simulink model "HybridShip_ModelE_PlantStepE_Stream"  (R2026a)
settings: Solver=ode3  StopTime=7200  FixedStep=0.01
undefined symbols (not defined in the file): ADAPTER_FORCE_MODE, ADAPTER_FORCE_P1_KW, ADAPTER_FORCE_P2_KW, ASSUMED_C_bus, ASSUMED_Drive_TimeConstant, ASSUMED_eta_dcdc, ASSUMED_eta_rect, ASSUMED_K_droop, ASSUMED_SOC_ChgDerate_Start, ASSUMED_SOC_DisDerate_Start, ASSUMED_SOC_max, ASSUMED_SOC_min, ASSUMED_SpeedPI_Ki, ASSUMED_SpeedPI_Kp, ASSUMED_V_floor, Bat_C1_LUT_F, Bat_eta_coul, Bat_I_limit_surrogate_A, Bat_OCV_LUT_V, Bat_P_conv_bus_max_kW, Bat_Q_nom_Ah, Bat_R0_chg_mult, Bat_R0_LUT_ohm, Bat_R1_LUT_ohm, Bat_SOC_init, Bat_SOC_LUT_nodes, Bat_V_max_V, Bat_V_min_V, CCS_Vdc_Steady_Band, CCS_Vdc_Transient_Band, DG_BSFC_gkWh, DG_BSFC_P_kW, DG_C_start_kg, DG_P_min_kW, DG_P_rated_kW, DG_ramp_kW_per_s, DG_t_starting_s, DG_t_sync_s, DG_tau_s, DiscIntNeverNeededParam, Elec_Eff, F_env_const, Gear_Eff, Gear_Ratio, Hull_k_form, Hull_K_R, Hull_Lpp_m, Hull_T_m, K_Fv, K_Fw, K_Qv, K_Qw, Manual_Cmd_RateLimit_kW_per_s, Mot_P_nom, Mot_T_max, N_ticks_cooldown, N_ticks_starting, N_ticks_sync, nu_water, omega_min_radps ... (+40)
libraries: simulink x6
(part 2 of 2)

== matlab function HybridShip_ModelE_PlantStepE_Stream/06_Genset_System/GensetUnitE_DG1 ==
  settings: updateMethod=DISCRETE  sampleTime=0.01
  data: cmd_start input; P_actual_kW output; cmd_stop input; P_ref_kW input; state output; below_min_flag output; start_count output; DG_P_rated_kW parameter; DG_P_min_kW parameter; DG_ramp_kW_per_s parameter; DG_tau_s parameter; N_ticks_starting parameter; N_ticks_sync parameter; N_ticks_cooldown parameter; Pgen_init parameter
function [P_actual_kW, state, below_min_flag, start_count] = GensetUnitE(...
    cmd_start, cmd_stop, P_ref_kW, ...
    DG_P_rated_kW, DG_P_min_kW, DG_ramp_kW_per_s, DG_tau_s, ...
N_ticks_starting, N_ticks_sync, N_ticks_cooldown, Pgen_init)
%#codegen
% GensetUnitE：单发电机组启停状态机 + 功率链（Model E, FR-418/419, OQ-6 定稿）
%   DG1/DG2 各用一个块实例（同一代码）；固定步 0.01 s，每步调用一次 = 1 tick；
%   状态驻留用整数 tick 计数做转移判据（OQ-6，禁止浮点时间比较）。
%   state: 0=OFF 1=STARTING 2=SYNCHRONIZING 3=ON 4=COOLDOWN（数值状态，供 fuel/log 用）
%   D-4：min up/min down time 不在本 Plant 内（unit commitment 属 B 包 PMS v2）；
%        COOLDOWN 物理驻留 N_ticks_cooldown 表达停机间隔，期间 cmd_start 忽略。
%   aborted-start：STARTING/SYNC 不可中断；cmd_stop 只置 pending_stop，进入 ON 后一拍内执行停机。
%   OFF 态 stop 优先（2026-09-04 主 Agent 裁决）：cmd_start=1 且 cmd_stop=1 时保持 OFF，防停机后无限再启动。
persistent st n_tick pending_stop n_starts P_ramp P_lag
if isempty(st)
    st = 0;                 % 初始 OFF（新状态机初始 OFF；Pgen_init 仅作 P_lag legacy 初值）
    n_tick = 0;             % 当前状态驻留 tick 计数
    pending_stop = false;   % STARTING/SYNC 期间登记的停机请求
    n_starts = 0;           % 完成启动次数（SYNC 完成时 +1，含 aborted-start）
    P_ramp = 0;             % 爬坡状态 [kW]
    P_lag = Pgen_init;      % 一阶惯性状态 [kW]（legacy 常开模型初值兼容语义）
end

P_actual_kW = 0;            % 非 ON 态恒 0；ON 态由功率链覆写
below_min_flag = 0;         % 仅 ON 态置位（ref < P_min；switch 后按最终状态统一判定）

switch st
    case 0 % OFF：cmd_start 触发启动（cmd_stop 有效时 stop 优先，防停机后无限再启动）
        if cmd_start > 0.5 && cmd_stop < 0.5
            st = 1;                  % OFF -> STARTING
            n_tick = 0;
            pending_stop = false;    % n_starts 不在此刻加（SYNC 完成时才计）
            P_ramp = 0;              % 启动从零爬坡
            P_lag = 0;
        end

    case 1 % STARTING：不可中断（aborted-start 只登记）
        n_tick = n_tick + 1;
        if cmd_stop > 0.5
            pending_stop = true;
        end
        if n_tick >= N_ticks_starting
            st = 2;                  % STARTING -> SYNCHRONIZING
            n_tick = 0;
        end

    case 2 % SYNCHRONIZING：不可中断
        n_tick = n_tick + 1;
        if cmd_stop > 0.5
            pending_stop = true;
        end
        if n_tick >= N_ticks_sync
            n_starts = n_starts + 1; % 启动完成（启动燃油由此计量一次）
            st = 3;                  % SYNCHRONIZING -> ON
            n_tick = 0;
        end

    case 3 % ON：功率链 + 停机命令（pending_stop 在此执行）
        if cmd_stop > 0.5 || pending_stop
            pending_stop = false;
            st = 4;                  % ON -> COOLDOWN（断路器分闸，本拍 P=0）
            n_tick = 0;
        else
            % ref clamp [P_min, rated]（below_min_flag 在 switch 后按最终状态统一置位）
            P_ref_c = min(max(P_ref_kW, DG_P_min_kW), DG_P_rated_kW);
            if P_ramp < P_ref_c
                P_ramp = min(P_ramp + DG_ramp_kW_per_s*0.01, P_ref_c);  % 爬坡限幅（0.01 s 步）
            elseif P_ramp > P_ref_c
                P_ramp = max(P_ramp - DG_ramp_kW_per_s*0.01, P_ref_c);
            end
            P_lag = P_lag + (P_ramp - P_lag)*0.01/DG_tau_s;             % 一阶惯性 tau
            P_actual_kW = min(max(P_lag, 0), DG_P_rated_kW);
            % 注：爬坡过渡期 P<P_min 为 registered 过渡（below_min_flag 登记；
            % 燃油侧按 clamp 到 BSFC 下节点(125)查表，见 FuelModelE）
        end

    case 4 % COOLDOWN：P=0；cmd_start 忽略（D-4：物理驻留表达最小停机间隔）
        n_tick = n_tick + 1;
        if n_tick >= N_ticks_cooldown
            st = 0;                  % COOLDOWN -> OFF
            n_tick = 0;
        end

    otherwise % 防御：非法状态归 OFF（无 NaN 路径）
        st = 0;
        n_tick = 0;
end

state = st;                  % 输出为本拍转移后的状态
if st == 3 && P_ref_kW < DG_P_min_kW
    below_min_flag = 1;      % 输出约定：flag=1 当且仅当 state==3 且 ref<P_min（含 ON 入口拍）
end
start_count = n_starts;
end

== matlab function HybridShip_ModelE_PlantStepE_Stream/06_Genset_System/GensetUnitE_DG2 ==
  settings: updateMethod=DISCRETE  sampleTime=0.01
  data: cmd_start input; P_actual_kW output; cmd_stop input; P_ref_kW input; state output; below_min_flag output; start_count output; DG_P_rated_kW parameter; DG_P_min_kW parameter; DG_ramp_kW_per_s parameter; DG_tau_s parameter; N_ticks_starting parameter; N_ticks_sync parameter; N_ticks_cooldown parameter; Pgen_init parameter
function [P_actual_kW, state, below_min_flag, start_count] = GensetUnitE(...
    cmd_start, cmd_stop, P_ref_kW, ...
    DG_P_rated_kW, DG_P_min_kW, DG_ramp_kW_per_s, DG_tau_s, ...
N_ticks_starting, N_ticks_sync, N_ticks_cooldown, Pgen_init)
%#codegen
% GensetUnitE：单发电机组启停状态机 + 功率链（Model E, FR-418/419, OQ-6 定稿）
%   DG1/DG2 各用一个块实例（同一代码）；固定步 0.01 s，每步调用一次 = 1 tick；
%   状态驻留用整数 tick 计数做转移判据（OQ-6，禁止浮点时间比较）。
%   state: 0=OFF 1=STARTING 2=SYNCHRONIZING 3=ON 4=COOLDOWN（数值状态，供 fuel/log 用）
%   D-4：min up/min down time 不在本 Plant 内（unit commitment 属 B 包 PMS v2）；
%        COOLDOWN 物理驻留 N_ticks_cooldown 表达停机间隔，期间 cmd_start 忽略。
%   aborted-start：STARTING/SYNC 不可中断；cmd_stop 只置 pending_stop，进入 ON 后一拍内执行停机。
%   OFF 态 stop 优先（2026-09-04 主 Agent 裁决）：cmd_start=1 且 cmd_stop=1 时保持 OFF，防停机后无限再启动。
persistent st n_tick pending_stop n_starts P_ramp P_lag
if isempty(st)
    st = 0;                 % 初始 OFF（新状态机初始 OFF；Pgen_init 仅作 P_lag legacy 初值）
    n_tick = 0;             % 当前状态驻留 tick 计数
    pending_stop = false;   % STARTING/SYNC 期间登记的停机请求
    n_starts = 0;           % 完成启动次数（SYNC 完成时 +1，含 aborted-start）
    P_ramp = 0;             % 爬坡状态 [kW]
    P_lag = Pgen_init;      % 一阶惯性状态 [kW]（legacy 常开模型初值兼容语义）
end

P_actual_kW = 0;            % 非 ON 态恒 0；ON 态由功率链覆写
below_min_flag = 0;         % 仅 ON 态置位（ref < P_min；switch 后按最终状态统一判定）

switch st
    case 0 % OFF：cmd_start 触发启动（cmd_stop 有效时 stop 优先，防停机后无限再启动）
        if cmd_start > 0.5 && cmd_stop < 0.5
            st = 1;                  % OFF -> STARTING
            n_tick = 0;
            pending_stop = false;    % n_starts 不在此刻加（SYNC 完成时才计）
            P_ramp = 0;              % 启动从零爬坡
            P_lag = 0;
        end

    case 1 % STARTING：不可中断（aborted-start 只登记）
        n_tick = n_tick + 1;
        if cmd_stop > 0.5
            pending_stop = true;
        end
        if n_tick >= N_ticks_starting
            st = 2;                  % STARTING -> SYNCHRONIZING
            n_tick = 0;
        end

    case 2 % SYNCHRONIZING：不可中断
        n_tick = n_tick + 1;
        if cmd_stop > 0.5
            pending_stop = true;
        end
        if n_tick >= N_ticks_sync
            n_starts = n_starts + 1; % 启动完成（启动燃油由此计量一次）
            st = 3;                  % SYNCHRONIZING -> ON
            n_tick = 0;
        end

    case 3 % ON：功率链 + 停机命令（pending_stop 在此执行）
        if cmd_stop > 0.5 || pending_stop
            pending_stop = false;
            st = 4;                  % ON -> COOLDOWN（断路器分闸，本拍 P=0）
            n_tick = 0;
        else
            % ref clamp [P_min, rated]（below_min_flag 在 switch 后按最终状态统一置位）
            P_ref_c = min(max(P_ref_kW, DG_P_min_kW), DG_P_rated_kW);
            if P_ramp < P_ref_c
                P_ramp = min(P_ramp + DG_ramp_kW_per_s*0.01, P_ref_c);  % 爬坡限幅（0.01 s 步）
            elseif P_ramp > P_ref_c
                P_ramp = max(P_ramp - DG_ramp_kW_per_s*0.01, P_ref_c);
            end
            P_lag = P_lag + (P_ramp - P_lag)*0.01/DG_tau_s;             % 一阶惯性 tau
            P_actual_kW = min(max(P_lag, 0), DG_P_rated_kW);
            % 注：爬坡过渡期 P<P_min 为 registered 过渡（below_min_flag 登记；
            % 燃油侧按 clamp 到 BSFC 下节点(125)查表，见 FuelModelE）
        end

    case 4 % COOLDOWN：P=0；cmd_start 忽略（D-4：物理驻留表达最小停机间隔）
        n_tick = n_tick + 1;
        if n_tick >= N_ticks_cooldown
            st = 0;                  % COOLDOWN -> OFF
            n_tick = 0;
        end

    otherwise % 防御：非法状态归 OFF（无 NaN 路径）
        st = 0;
        n_tick = 0;
end

state = st;                  % 输出为本拍转移后的状态
if st == 3 && P_ref_kW < DG_P_min_kW
    below_min_flag = 1;      % 输出约定：flag=1 当且仅当 state==3 且 ref<P_min（含 ON 入口拍）
end
start_count = n_starts;
end

== matlab function HybridShip_ModelE_PlantStepE_Stream/07_PMS_v2/PMS_Demand_Policy ==
  settings: updateMethod=DISCRETE  sampleTime=0.01
  data: P_load_gen_kW input; P_gen_req_baseline_kW output; SOC input; N_dispatch_fb input; P_commit_kW output; u_recovery output; P_recovery_actual_kW output; PMS_LoadLPF_tau_s parameter double size=1; PMS_SOC_lo parameter double size=1; PMS_SOC_recovered parameter double size=1; PMS_P_chg_recovery_kW parameter double size=1; DG_P_rated_kW parameter double size=1
function [P_gen_req_baseline_kW, P_commit_kW, u_recovery, P_recovery_actual_kW] = PMSDemandPolicyE(P_load_gen_kW, SOC, N_dispatch_fb, PMS_LoadLPF_tau_s, PMS_SOC_lo, PMS_SOC_recovered, PMS_P_chg_recovery_kW, DG_P_rated_kW)
%#codegen
% PMSDemandPolicyE：Baseline_Demand_Policy 发电需求律（Model E Phase 4-B, FR-432~435, T-002 链 A）
%   依据：.specs/phase4-b-pms-safety/design.md §5.3 + requirements FR-432/433/434/435（AC-417）；
%   brainstorm D-B3（Demand Policy 四数冻结）/ D-B4（P_commit 信号语义方案 b）/ D-B6 / D-B14。
%   角色：07_PMS_v2 内 Baseline source（ems_health_ok=0 时的确定性热备份，D-B7 ③）；
%   advanced EMS source 的 P_gen_req=P_EMS 直送不削减（FR-434），削减只发生在本 Baseline source 内部。
%
%   canonical 功率域（DD-1，genset-side generator-equivalent）：
%     - 全部输入/输出量均为 genset-side generator-equivalent；P_load_gen_kW 已在 07_PMS_v2
%       输入边界经 X_b2g_* 由 bus 侧 ÷ASSUMED_eta_rect 换算入域，本块零换算直用；
%     - PMS_P_chg_recovery_kW=100 kW 为 generator-equivalent recovery bias（≈bus 侧新增发电
%       约 97 kW），禁止表述为"电池 100 kW 实际充电"（DD-1 措辞纪律）。
%
%   输入：P_load_gen_kW 负荷（generator-equivalent）；SOC [-]；N_dispatch_fb dispatch 反馈
%     （在线机组数，**上一拍语义由调用方 UnitDelay 保证**——本函数直接消费当拍入参，
%     内部不再延迟，design §5.3）；PMS_LoadLPF_tau_s / PMS_SOC_lo / PMS_SOC_recovered /
%     PMS_P_chg_recovery_kW 为 FR-435 四参数（全 ENGINEERING_SURROGATE，数值事实源
%     config/ModelE_Control_Parameters.m，敏感性 τ∈{30,120} 冻结登记不扫）；DG_P_rated_kW
%     单机额定（genset 域字面，DD-1）。
%   输出：P_gen_req_baseline_kW = LPF(P_load) + P_recovery_actual（FR-432）；
%     P_commit_kW = LPF(P_load)（commitment 判据信号，不含 recovery 偏置，D-B4 方案 b）；
%     u_recovery SOC 滞回状态（供 logging，design §5.3）；P_recovery_actual_kW 实际恢复偏置。
%
%   离散约定：固定步 0.01 s，每调用一次 = 1 tick；dt=0.01 硬编码于 LPF 更新，
%   若模型固定步长变更须一并重推（同 GensetUnitE OQ-6 口径）。
%   纯 MATLAB：persistent 为唯一状态载体；无 toolbox 依赖；无 evalin/assignin/全局变量。

persistent P_load_filt u_rec
% 注：R2026a MATLAB Function 块解析纪律——persistent 变量不得直接作为输出参量，
% 故滞回状态本体为 u_rec，输出名 u_recovery 在每拍末拷贝输出（语义不变）。
if isempty(P_load_filt)
    P_load_filt = P_load_gen_kW;    % y[0]=x[0]（design §5.3；首拍 LPF 更新数值恒等）
    u_rec = false;                  % FR-433 初值 false
end

% (1) 一阶 LPF 前向欧拉（FR-432）：y[k]=y[k-1]+(Ts/τ)(x[k]-y[k-1])，τ=PMS_LoadLPF_tau_s
%     前向欧拉**非双线性**；标称 τ=60 s 时 Ts/τ≈1.67e-4，远在 0<Ts/τ<2 稳定界内、稳定裕量大
%     （禁称"无条件稳定"，design §5.3 措辞纪律）。
P_load_filt = P_load_filt + (0.01/PMS_LoadLPF_tau_s)*(P_load_gen_kW - P_load_filt);

% (2) SOC 滞回（FR-433，比较符号冻结；D-B3）：<=PMS_SOC_lo 进 / >=PMS_SOC_recovered 出 / 其间保持
if SOC <= PMS_SOC_lo
    u_rec = true;
elseif SOC >= PMS_SOC_recovered
    u_rec = false;
end
u_recovery = u_rec;                 % 输出本拍评估后的滞回状态（供 logging，design §5.3）

% (3) 恢复偏置（FR-434 non-firm/opportunistic）：负荷服务优先，削减只在 Baseline source 内部
%     （recovery 不得单独触发 DG2 启动——commitment 判据用 P_commit_kW，D-B4 结构性规则；
%       EMS 直送不削减，指令/功率 mismatch 经 dispatch 诊断量暴露，D-B6/D-B14）
P_recovery_actual_kW = double(u_rec) * max(0, min(PMS_P_chg_recovery_kW, ...
    DG_P_rated_kW*N_dispatch_fb - P_load_filt));

% (4) 基线发电需求 = LPF(P_load) + 实际恢复偏置（FR-432 / design §5.3）
P_gen_req_baseline_kW = P_load_filt + P_recovery_actual_kW;

% (5) commitment 判据信号 = LPF(P_load)，不含 recovery 偏置（D-B4 方案 b：
%     恢复充电为 opportunistic/non-firm 需求，不得影响启停门槛判定）
P_commit_kW = P_load_filt;
end

== stateflow chart HybridShip_ModelE_PlantStepE_Stream/07_PMS_v2/PMS_Commitment_Supervisor ==
  settings: updateMethod=DISCRETE  sampleTime=0.01
  state ONE_DG_NORMAL
    entry: if (commitment_state == 0)
    commitment_state = 1;
    reason_code = 0;
    audit_valid = 0;
    start_hold_timer = 0; stop_hold_timer = 0; online_timer = 0;
    cmd_onoff_DG1 = double(fault_latch_DG1 < 0.5);
    cmd_onoff_DG2 = 0;
    else
    audit_old_state = commitment_state; audit_new_state = 1;
    audit_P_commit_kW = P_commit_kW;
    audit_t_start_hold = start_hold_timer; audit_t_stop_hold = stop_hold_timer;
    audit_t_online = online_timer;
    audit_safety_override = double(tr_reason >= 3);
    audit_valid = 1;
    reason_code = tr_reason;
    commitment_state = 1;
    start_hold_timer = 0; stop_hold_timer = 0; online_timer = 0;
    cmd_onoff_DG1 = double(fault_latch_DG1 < 0.5);
    cmd_onoff_DG2 = 0;
    end
    during: cmd_onoff_DG1 = double(fault_latch_DG1 < 0.5);
    cmd_onoff_DG2 = 0;
    stop_hold_timer = 0; online_timer = 0;
    if (P_commit_kW > PMS_start_threshold_kW)
    start_hold_timer = min(start_hold_timer + 1, T_start_hold_ticks);
    else
    start_hold_timer = 0;
    end
  state DG2_START_PENDING
    entry: audit_old_state = commitment_state; audit_new_state = 2;
    audit_P_commit_kW = P_commit_kW;
    audit_t_start_hold = start_hold_timer; audit_t_stop_hold = stop_hold_timer;
    audit_t_online = online_timer;
    audit_safety_override = double(tr_reason >= 3);
    audit_valid = 1;
    reason_code = tr_reason; pending_reason = tr_reason;
    commitment_state = 2;
    start_hold_timer = 0; stop_hold_timer = 0; online_timer = 0;
    cmd_onoff_DG1 = double(fault_latch_DG1 < 0.5);
    cmd_onoff_DG2 = double(fault_latch_DG2 < 0.5);
    during: cmd_onoff_DG1 = double(fault_latch_DG1 < 0.5);
    cmd_onoff_DG2 = double(fault_latch_DG2 < 0.5);
    start_hold_timer = 0; stop_hold_timer = 0; online_timer = 0;
  state TWO_DG_NORMAL
    entry: audit_old_state = commitment_state; audit_new_state = 3;
    audit_P_commit_kW = P_commit_kW;
    audit_t_start_hold = start_hold_timer; audit_t_stop_hold = stop_hold_timer;
    audit_t_online = online_timer;
    audit_safety_override = double(tr_reason >= 3);
    audit_valid = 1;
    reason_code = tr_reason;
    commitment_state = 3;
    start_hold_timer = 0; stop_hold_timer = 0; online_timer = 0;
    cmd_onoff_DG1 = double(fault_latch_DG1 < 0.5);
    cmd_onoff_DG2 = double(fault_latch_DG2 < 0.5);
    during: cmd_onoff_DG1 = double(fault_latch_DG1 < 0.5);
    cmd_onoff_DG2 = double(fault_latch_DG2 < 0.5);
    start_hold_timer = 0;
    if (P_commit_kW < PMS_stop_threshold_kW)
    stop_hold_timer = min(stop_hold_timer + 1, T_stop_hold_ticks);
    else
    stop_hold_timer = 0;
    end
    if (state_DG2 == 3)
    online_timer = min(online_timer + 1, PMS_min_up_ticks);
    else
    online_timer = 0;
    end
  DG2_START_PENDING -> ONE_DG_NORMAL [order 1] : [fault_latch_DG2 > 0.5]{tr_reason = 3;}
  TWO_DG_NORMAL -> ONE_DG_NORMAL [order 1] : [fault_latch_DG2 > 0.5]{tr_reason = 3;}
  TWO_DG_NORMAL -> ONE_DG_NORMAL [order 2] : [force_stop_dg2_req > 0.5]{tr_reason = force_stop_reason;}
  TWO_DG_NORMAL -> ONE_DG_NORMAL [order 3] : [P_commit_kW < PMS_stop_threshold_kW && stop_hold_timer >= T_stop_hold_ticks && online_timer >= PMS_min_up_ticks]{tr_reason = 2;}
  (default) -> ONE_DG_NORMAL : {tr_reason = 0;}
  ONE_DG_NORMAL -> DG2_START_PENDING [order 1] : [force_start_dg2_req > 0.5 && fault_latch_DG2 < 0.5]{tr_reason = force_start_reason;}
  ONE_DG_NORMAL -> DG2_START_PENDING [order 2] : [start_hold_timer >= T_start_hold_ticks && fault_latch_DG2 < 0.5]{tr_reason = 1;}
  DG2_START_PENDING -> TWO_DG_NORMAL [order 2] : [state_DG2 == 3]{tr_reason = pending_reason;}
  data: P_commit_kW input double size=1; state_DG2 input double size=1; fault_latch_DG1 input double size=1; fault_latch_DG2 input double size=1; force_start_dg2_req input double size=1; force_start_reason input double size=1; force_stop_dg2_req input double size=1; force_stop_reason input double size=1; cmd_onoff_DG1 output double size=1 =0; cmd_onoff_DG2 output double size=1 =0; commitment_state output double size=1 =0; reason_code output double size=1 =0; start_hold_timer output double size=1 =0; stop_hold_timer output double size=1 =0; online_timer output double size=1 =0; audit_valid output double size=1 =0; audit_old_state output double size=1 =0; audit_new_state output double size=1 =0; audit_P_commit_kW output double size=1 =0; audit_t_start_hold output double size=1 =0; audit_t_stop_hold output double size=1 =0; audit_t_online output double size=1 =0; audit_safety_override output double size=1 =0; tr_reason local double size=1 =0; pending_reason local double size=1 =0; PMS_start_threshold_kW parameter double size=1; PMS_stop_threshold_kW parameter double size=1; T_start_hold_ticks parameter double size=1; T_stop_hold_ticks parameter double size=1; PMS_min_up_ticks parameter double size=1

== matlab function HybridShip_ModelE_PlantStepE_Stream/07_PMS_v2/PMS_Dispatch_Allocator ==
  data: P_gen_req_eff_kW input; P_DG1_ref_kW output; state_DG1 input; state_DG2 input; dispatch_eligible_DG1 input; dispatch_eligible_DG2 input; P_DG2_ref_kW output; N_dispatch output; P_gen_unserved_kW output; P_gen_surplus_kW output; dispatch_min_clamp_active output; dispatch_n_zero_flag output; DG_P_min_kW parameter double size=1; DG_P_rated_kW parameter double size=1
function [P_DG1_ref_kW, P_DG2_ref_kW, N_dispatch, P_gen_unserved_kW, P_gen_surplus_kW, dispatch_min_clamp_active, dispatch_n_zero_flag] = PMSDispatchAllocatorE(P_gen_req_eff_kW, state_DG1, state_DG2, dispatch_eligible_DG1, dispatch_eligible_DG2, DG_P_min_kW, DG_P_rated_kW)
%#codegen
% PMSDispatchAllocatorE：DG_Dispatch_Allocator 均分分配器（Model E, FR-441/442/443）
%   依据：design.md §5.5（is_dispatching 单一谓词，D-B15）+ §2 裁决③ + D-B6（分配律冻结）
%   + DD-1（canonical 域 = genset-side，dispatch 输出直连 Plant 零换算）。
%   采样约定：固定步 0.01 s，每调用一次 = 1 tick；本块为组合逻辑（无 persistent 状态，
%   state/eligible 输入均为 Commitment/fault 裁决后当拍值），dt 仅作口径登记——
%   若模型固定步长变更须一并重推（同 GensetUnitE OQ-6 口径）。
%   机组状态枚举（A2 GensetUnitE 口径）：0=OFF 1=STARTING 2=SYNCHRONIZING 3=ON 4=COOLDOWN。
%
%   is_dispatching 单一谓词（D-B15）：分母与输出共用同一谓词，禁止分母查 state 而
%   输出只查 eligible 的分裂写法（分裂可致 STARTING 机组获得非零 ref，违反 A2 契约）：
%       is_dispatching_i = (state_i==ON) ∧ dispatch_eligible_i；
%   STARTING/SYNC/COOLDOWN/OFF 对 N_dispatch 的贡献必为 0。
%
%   语义红线 a（A2 不得虚构输出功率契约）：STARTING/SYNC/COOLDOWN 机组即使
%   healthy∧available 也必须 ref==0（单测必含 STARTING+healthy+available ⇒ P_ref==0 case）。
%   语义红线 b（D-B14）：P_gen_unserved_kW 为 generation-command mismatch 纯诊断量
%   （EMS 过度请求≠真实缺口），禁用于 Safety 判据——S2 实际缺口判据用 realized
%   supply deficit 口径（design §5.6）。
%   语义红线 c（design §2 裁决③）：dispatch_min_clamp_active 为控制器意图语义
%   （is_dispatching ∧ P_raw<DG_P_min，严格小于），与 Plant below_min_flag
%   （state==3 && P_ref_kW<DG_P_min_kW 的意图口径，A2 GensetUnitE 输出约定）区分。
%
%   DISPATCH_MODE 登记（FR-443/D-B1，仅注释与接口文档，不写第二模式代码分支）：
%       0=AGGREGATE_AUTO（本块实现）/ 1=EXTERNAL_PER_UNIT（reserved）。
%   禁止 BSFC-aware 分配、不对称加载与轮换——DG1=lead / DG2=lag 固定对称均分
%   （D-B6 冻结，equal-rated parallel gensets under symmetric load-sharing configuration）。
%   N_dispatch==0 为防御分支（voyage active 期间不应发生，v1 无 0DG 基线假设）：
%   双机 ref=0 + dispatch_n_zero_flag=1，不虚构功率、不静默吞掉请求。
%
%   参数纪律：DG_P_min_kW / DG_P_rated_kW 全部经入参传入（数值事实源
%   config/ModelE_Physics_Parameters.m §5，禁止在此写死或重议）。

dt = 0.01;  % [s] 离散步长登记（每调用一次 = 1 tick）；本块无时间积分，dt 仅口径声明——若模型固定步长变更须一并重推（同 GensetUnitE OQ-6 口径）

% ---- is_dispatching 单一谓词（分母与输出共用同一谓词，D-B15）----
is1 = (state_DG1 == 3) && (dispatch_eligible_DG1 > 0.5);  % 3=ON 且裁决后 eligible 才参与
is2 = (state_DG2 == 3) && (dispatch_eligible_DG2 > 0.5);  % STARTING/SYNC/COOLDOWN/OFF 必排除
N_dispatch = double(is1) + double(is2);                   % 参与均分的机组数

% ---- 输出初值（N=0 防御分支语义：ref=0、surplus=0、min_clamp=0、unserved=max(0,req−0)）----
P_DG1_ref_kW = 0;
P_DG2_ref_kW = 0;
P_gen_unserved_kW  = max(0, P_gen_req_eff_kW);   % ΣP_i_ref=0 → unserved=max(0,req)
P_gen_surplus_kW   = 0;
dispatch_min_clamp_active = 0;
dispatch_n_zero_flag = 0;

if N_dispatch == 0
    % 防御：N_dispatch==0（不应发生于 voyage active）——flag 显式暴露，不虚构功率
    dispatch_n_zero_flag = 1;
else
    % ---- 均分 + clamp（FR-441/D-B6：P_i,ref = clamp(P_gen_req_eff/N_dispatch, P_min, P_max)）----
    P_raw = P_gen_req_eff_kW / N_dispatch;
    if is1
        P_DG1_ref_kW = min(max(P_raw, DG_P_min_kW), DG_P_rated_kW);
    end
    if is2
        P_DG2_ref_kW = min(max(P_raw, DG_P_min_kW), DG_P_rated_kW);
    end
    % ---- 诊断三件套（FR-442）----
    P_sum = P_DG1_ref_kW + P_DG2_ref_kW;
    P_gen_unserved_kW = max(0, P_gen_req_eff_kW - P_sum);  % 红线 b：纯诊断，禁用于 Safety 判据
    P_gen_surplus_kW  = max(0, P_sum - P_gen_req_eff_kW);
    % 红线 c：控制器意图语义——任一参与机组 P_raw 低于 P_min（严格小于，等号不触发）
    if (is1 && (P_raw < DG_P_min_kW)) || (is2 && (P_raw < DG_P_min_kW))
        dispatch_min_clamp_active = 1;
    end
end
end

== matlab function HybridShip_ModelE_PlantStepE_Stream/16_Safety_Interlock/PMS_Safety_Interlock ==
  settings: updateMethod=DISCRETE  sampleTime=0.01
  data: state_DG1 input; force_start_req output size=[1 2]; state_DG2 input; cmd_onoff_1 input; cmd_onoff_2 input; P_load_gen_kW input; P_prop_dem_kW input; P_hotel_kW input; P_DG1_kW input; P_DG2_kW input; P_bat_dis_avail_g_kW input; P_bat_chg_avail_g_kW input; N_dispatch input; SOC input; Vdc_V input; bat_flag_1 input; bat_flag_2 input; bat_flag_3 input; P_gen_ref_kW input; ems_health_raw input; nominal_is_ems input; voyage_active input; force_start_reason output size=1; force_stop_req output size=[1 2]; force_stop_reason output size=1; fault_latch output size=[1 2]; ems_health_ok output size=1; baseline_fallback_active output size=1; baseline_fallback_reason output size=1; min_gen_surplus_unresolved output size=1; D_firm_kW output size=1; S2_supply_gap_kW output size=1; flag_soc_low output size=1; flag_vdc_low output size=1; flag_bat_passthrough output size=[1 3]; PMS_S2_hold_ticks parameter double size=1; PMS_S4_hold_ticks parameter double size=1; PMS_start_fail_ticks parameter double size=1; PMS_firm_margin_kW parameter double size=1; DG_P_rated_kW parameter double size=1; DG_P_min_kW parameter double size=1; ASSUMED_eta_rect parameter double size=1
function [force_start_req, force_start_reason, force_stop_req, force_stop_reason, fault_latch, ems_health_ok, baseline_fallback_active, baseline_fallback_reason, min_gen_surplus_unresolved, D_firm_kW, S2_supply_gap_kW, flag_soc_low, flag_vdc_low, flag_bat_passthrough] = PMSSafetyInterlockE(state_DG1, state_DG2, cmd_onoff_1, cmd_onoff_2, P_load_gen_kW, P_prop_dem_kW, P_hotel_kW, P_DG1_kW, P_DG2_kW, P_bat_dis_avail_g_kW, P_bat_chg_avail_g_kW, N_dispatch, SOC, Vdc_V, bat_flag_1, bat_flag_2, bat_flag_3, P_gen_ref_kW, ems_health_raw, nominal_is_ems, voyage_active, PMS_S2_hold_ticks, PMS_S4_hold_ticks, PMS_start_fail_ticks, PMS_firm_margin_kW, DG_P_rated_kW, DG_P_min_kW, ASSUMED_eta_rect)
%#codegen
% PMSSafetyInterlockE —— 16_Safety_Interlock 安全联锁（Model E, FR-444/445/446/447, design §5.6 评审修订版）
%   离散步长约定：每调用一次 = 1 tick = 0.01 s；dt=0.01 硬编码于全部 tick 计数口径，
%   若模型固定步长变更须一并重推（同 GensetUnitE OQ-6 口径）。
%   职责边界（FR-444 / design §5.6 / §5.7）：
%     (1) 16 号不直写 Plant——override 请求总线经 UnitDelay（0.01 s）回 07_PMS_v2 作
%         Commitment Supervisor / source selector 高优先级输入；本函数本体不管 UnitDelay，
%         一拍拍序断言（override(t) ⇒ t+0.01 s 恰好一拍到达、无代数环）移交集成层 T-007；
%     (2) 08_Undervolt_Derate 保持唯一执行性 propulsion limiter，本函数无推进限制输出
%         （与 08 无任何信号直连，两者作用通道完全分离，FR-446/design §5.7）；
%     (3) fault_latch 锁存至仿真结束：v1 无 run 内复位通道，登记 future extension（D-B11）。
%   机组状态枚举（同链 B GensetUnitE）：0=OFF 1=STARTING 2=SYNCHRONIZING 3=ON 4=COOLDOWN。
%   reason 枚举（force_start_reason / force_stop_reason）：
%     0=无 3=SAFETY_DG_FAULT 4=SAFETY_REALIZED_SUPPLY_DEFICIT
%     5=SAFETY_PROSPECTIVE_FIRM_CAPACITY_DEFICIT 6=SAFETY_MIN_GEN_SURPLUS。
%   baseline_fallback_reason 枚举：0=无 1=健康通道失效 2=P_gen_ref 非有限。
%   域约定（DD-1，canonical 域 = genset-side）：全部比较量在 genset 域；P_bat_*_avail_g 与
%   P_load_gen 已由 07 边界换算，本函数只做算术、不做 ÷η_rect 域转换；S4 的
%   (P_prop_dem+P_hotel)/ASSUMED_eta_rect 是 design §5.6 公式自身的组成部分（bus 侧
%   commanded demand → genset 域 firm-capacity 要求），不算域转换点。
%   输出向量约定：force_start_req/force_stop_req/fault_latch [1×2]（DG1,DG2）；
%   flag_bat_passthrough [1×3]；全 override/flag 事件经输出端口入日志（VI-1，D-B7）。
persistent fl_latch prev_state s2_cnt s4_cnt s1b_ticks prev_fstp fback_active fback_reason min_srp
if isempty(fl_latch)
    fl_latch = zeros(1,2);    % S1 故障锁存（锁存至仿真结束，v1 无 run 内复位，D-B11 登记 future extension）
    prev_state = zeros(1,2);  % 上一拍机组状态（S1a 判据用）
    s2_cnt = 0;               % S2 连续判据计数 [tick]
    s4_cnt = 0;               % S4 连续判据计数 [tick]
    s1b_ticks = zeros(1,2);   % S1b STARTING/SYNC 连续驻留计数 [tick]
    prev_fstp = zeros(1,2);   % 上一拍 force_stop_req（S1a 判据用）
    fback_active = 0;         % S5 baseline fallback 锁存（D-B11：v1 不自动恢复）
    fback_reason = 0;         % S5 首因锁定事件码（1=通道失效 2=ref 非有限）
    min_srp = 0;              % S3 单健康机 unresolved 锁存（FR-445 S3 known out-of-scope）
end

st = [state_DG1, state_DG2];
cmd = [cmd_onoff_1, cmd_onoff_2];
P_DG = [P_DG1_kW, P_DG2_kW];

% ---- S1 DG fault 检测（design §5.6，D-B7 修正后语义，非字面 state≠command）----
% 先于 override 计算并用上一拍 prev_state/prev_fstp 判定，避免拍内自反馈。
for i = 1:2
    % S1a 非预期丢失：自非 OFF 进入 OFF/COOLDOWN ∧ cmd_onoff==1 ∧ 无本方 force_stop 在令
    if prev_state(i) ~= 0 && (st(i) == 0 || st(i) == 4) && cmd(i) > 0.5 && prev_fstp(i) < 0.5
        fl_latch(i) = 1;
    end
    % S1b 启动失败：state∈{STARTING,SYNC} 连续计数（否则清零），≥ PMS_start_fail_ticks → 锁存
    if st(i) == 1 || st(i) == 2
        s1b_ticks(i) = min(s1b_ticks(i) + 1, PMS_start_fail_ticks);  % 封顶防溢出，判据不变
        if s1b_ticks(i) >= PMS_start_fail_ticks
            fl_latch(i) = 1;
        end
    else
        s1b_ticks(i) = 0;
    end
end

% 健康在线机组数（S3/S4 共用口径：state==3 且未锁存故障；STARTING/SYNC 不计入，design §5.6）
n_on_healthy = 0;
for i = 1:2
    if st(i) == 3 && fl_latch(i) < 0.5
        n_on_healthy = n_on_healthy + 1;
    end
end

% ---- S2 Realized supply deficit（design §5.6 评审重定义，D-B14）----
% gap = max(0, P_load_gen − ΣP_DGi_actual)：判据基于实际供电能力而非指令错配；
% P_gen_unserved（generation-command mismatch）仅为 Dispatch 诊断量，禁用作本判据
% （design 反例：EMS 过度请求 800 kW 而实际负荷 300 kW 时 unserved>0 但无真实缺口）。
gap = P_load_gen_kW - (P_DG(1) + P_DG(2));
if gap < 0
    gap = 0;
end
S2_supply_gap_kW = gap;
if gap > P_bat_dis_avail_g_kW
    s2_cnt = min(s2_cnt + 1, PMS_S2_hold_ticks);  % 连续计数（封顶防溢出，判据不变）
else
    s2_cnt = 0;
end
s2_trig = s2_cnt >= PMS_S2_hold_ticks;

% ---- S4 Prospective firm-capacity deficit（design §5.6 公式，FR-445 S4）----
% P_load_req_gen = (P_prop_dem + P_hotel)/ASSUMED_eta_rect：÷η_rect 是 §5.6 公式自身
% 组成部分（见文件头域约定注释，DD-1）；firm_avail 只计 ON 健康机组（STARTING/SYNC 不计入）。
% S4 是 capacity adequacy 判据，不是 instantaneous ramp adequacy（ramp/τ 瞬态缺口归
% battery/S2/Vdc 链，design §5.6）。
P_load_req_gen = (P_prop_dem_kW + P_hotel_kW) / ASSUMED_eta_rect;
firm_avail = n_on_healthy * DG_P_rated_kW + P_bat_dis_avail_g_kW;
D_firm_kW = P_load_req_gen + PMS_firm_margin_kW - firm_avail;
if D_firm_kW > 0
    s4_cnt = min(s4_cnt + 1, PMS_S4_hold_ticks);
else
    s4_cnt = 0;
end
s4_trig = s4_cnt >= PMS_S4_hold_ticks;

% ---- S3 Min generation surplus（FR-445 S3，design §5.6）----
surplus_margin = N_dispatch * DG_P_min_kW - P_load_gen_kW;
s3_cond = surplus_margin > P_bat_chg_avail_g_kW;

% ---- S5 EMS health fallback（design §5.6，D-B15 显式通道口径）----
% ems_health_ok = 显式健康通道有效 ∧ isfinite(P_gen_ref_kW)；isfinite 覆盖 NaN/±Inf，
% 对健康通道本身也做 isfinite 防御；不做 temporal freeze inference（D-B11/D-B15：
% legacy 变体可合法长时输出常数，常值输出≠控制器死亡，freeze/heartbeat 契约待 F 包定义）。
raw_ok = (ems_health_raw > 0.5) && isfinite(ems_health_raw);
ems_health_ok = 0;
if raw_ok && isfinite(P_gen_ref_kW)
    ems_health_ok = 1;
end
% 仅当 nominal source==EMS_AGGREGATE 时 S5 产生 fallback（BASELINE_POLICY 模式下
% selector 本不消费 EMS 输出，健康恶化为非事件：不置位、不报警）；
% fallback 锁存不自动恢复（D-B11），fallback_reason 首因锁定。
if ems_health_ok < 0.5 && nominal_is_ems > 0.5
    if fback_active < 0.5
        fback_active = 1;
        if raw_ok
            fback_reason = 2;   % P_gen_ref 非有限
        else
            fback_reason = 1;   % 健康通道失效（含 raw 非有限）
        end
    end
end

% ---- force_start 目标选择（确定性：available∧healthy∧offline）----
% target_i = state_i==0 且 fault_latch_i<0.5；COOLDOWN(4) 不可作目标（Plant 忽略启动指令）。
tgt = zeros(1,2);
for i = 1:2
    if st(i) == 0 && fl_latch(i) < 0.5
        tgt(i) = 1;
    end
end

% ---- force_start 请求（优先级 S1 响应 > S2 > S4；同拍 S2、S4 同时触发 reason 取 4）----
fs_req = zeros(1,2);
fs_reason = 0;
% S1 响应：机组 i 故障锁存 → 另一机 j 满足 voyage_active∧target_j → force_start（reason=3）
if fl_latch(1) > 0.5 && voyage_active > 0.5 && tgt(2) > 0.5
    fs_req(2) = 1;
    fs_reason = 3;
end
if fl_latch(2) > 0.5 && voyage_active > 0.5 && tgt(1) > 0.5
    fs_req(1) = 1;
    fs_reason = 3;
end
% S2 触发：优先 DG2（target_2），否则 DG1（target_1）；无目标 → 请求=0（flag-only，
% 缺口仍由 S2_supply_gap_kW 记录）
if s2_trig
    if tgt(2) > 0.5
        if fs_req(2) < 0.5
            fs_req(2) = 1;
            if fs_reason == 0
                fs_reason = 4;
            end
        end
    elseif tgt(1) > 0.5
        if fs_req(1) < 0.5
            fs_req(1) = 1;
            if fs_reason == 0
                fs_reason = 4;
            end
        end
    end
end
% S4 触发：同目标逻辑（reason=5；双机 ON 或无可启机组 → flag-only）
if s4_trig
    if tgt(2) > 0.5
        if fs_req(2) < 0.5
            fs_req(2) = 1;
            if fs_reason == 0
                fs_reason = 5;
            end
        end
    elseif tgt(1) > 0.5
        if fs_req(1) < 0.5
            fs_req(1) = 1;
            if fs_reason == 0
                fs_reason = 5;
            end
        end
    end
end

% ---- force_stop 请求（S1 防御性 FORCE_STOP 故障机 reason=3；S3 触发 FORCE_STOP DG2
%      reason=6；同拍时 reason 取 3——veto 最高优先级）----
fstp_req = zeros(1,2);
fstp_reason = 0;
if fl_latch(1) > 0.5
    fstp_req(1) = 1;
    fstp_reason = 3;
end
if fl_latch(2) > 0.5
    fstp_req(2) = 1;
    fstp_reason = 3;
end
if s3_cond
    if n_on_healthy >= 2
        fstp_req(2) = 1;   % 停 lag 机 DG2（旁路 dwell 由 Commitment 处理，design §5.6 S3）
        if fstp_reason == 0
            fstp_reason = 6;
        end
    else
        % 条件成立但仅单健康在线机：禁止 force_stop（FR-445 S3 + FR-439 N_DG_on≥1，
        % 单健康机不得造成 0DG）→ flag-only 并登记 known out-of-scope condition。
        min_srp = 1;
    end
end

% ---- 纯监视 flag（FR-446：flag 入日志、不独立动作；阈值 spec 字面冻结）----
flag_soc_low = 0;
if SOC <= 0.20
    flag_soc_low = 1;
end
flag_vdc_low = 0;
if Vdc_V < 600
    flag_vdc_low = 1;
end
flag_bat_passthrough = zeros(1,3);
if bat_flag_1 > 0.5
    flag_bat_passthrough(1) = 1;
end
if bat_flag_2 > 0.5
    flag_bat_passthrough(2) = 1;
end
if bat_flag_3 > 0.5
    flag_bat_passthrough(3) = 1;
end

% ---- 输出与拍序状态更新 ----
force_start_req = fs_req;
force_start_reason = fs_reason;
force_stop_req = fstp_req;
force_stop_reason = fstp_reason;
fault_latch = fl_latch;
baseline_fallback_active = fback_active;
baseline_fallback_reason = fback_reason;
min_gen_surplus_unresolved = min_srp;
prev_fstp = fstp_req;   % 供下一拍 S1a 判定"无 force_stop 在令"
prev_state = st;        % 供下一拍 S1a 判定"自非 OFF"
end

== matlab function HybridShip_ModelE_PlantStepE_Stream/14_Battery_Converter/battery_ecm ==
  settings: updateMethod=DISCRETE  sampleTime=0.01
  data: P_droop_kW input; P_bat_bus_kW output; SOC input; dt input; Bat_SOC_LUT_nodes input; Bat_OCV_LUT_V input; Bat_R0_LUT_ohm input; Bat_R1_LUT_ohm input; Bat_C1_LUT_F input; Bat_R0_chg_mult input; Bat_eta_coul input; Bat_Q_nom_Ah input; Bat_V_min_V input; Bat_V_max_V input; Bat_I_limit_surrogate_A input; Bat_P_conv_bus_max_kW input; eta_dcdc input; SOC_min input; SOC_max input; SOC_DisDerate_Start input; SOC_ChgDerate_Start input; SOC_out output; V_bat_V output; I_bat_A output; dSOC_dt output; P_dis_avail_kW output; P_chg_avail_kW output; battery_power_limited output; battery_discriminant_limit output; ecm_lut_boundary_flag output
function [P_bat_bus_kW, SOC_out, V_bat_V, I_bat_A, dSOC_dt, ...
          P_dis_avail_kW, P_chg_avail_kW, battery_power_limited, ...
          battery_discriminant_limit, ecm_lut_boundary_flag] = BatteryECM(...
    P_droop_kW, SOC, dt, ...
    Bat_SOC_LUT_nodes, Bat_OCV_LUT_V, Bat_R0_LUT_ohm, Bat_R1_LUT_ohm, Bat_C1_LUT_F, ...
    Bat_R0_chg_mult, Bat_eta_coul, Bat_Q_nom_Ah, Bat_V_min_V, Bat_V_max_V, ...
    Bat_I_limit_surrogate_A, Bat_P_conv_bus_max_kW, eta_dcdc, ...
    SOC_min, SOC_max, SOC_DisDerate_Start, SOC_ChgDerate_Start)
%#codegen
% BatteryECM — LFP 1RC 等效电路模型 + SOP 四约束（T-008/T-009 链 C）
% design.md §4.5/§4.6 + OQ-9 冻结项；0.01 s 离散步进（与模型 fixed-step 一致）。
% 符号约定（FR-423）：I > 0 = 放电，P_bat_bus_kW > 0 = 向母线放电。
% E = OCV - V_1 与 V_1 均为状态量估计，无代数环（NFR-409）。
% dSOC_dt 交外部 Integrator（限幅 [SOC_min, SOC_max] = [0.10, 0.95]）。
% Bat_eta_coul 仅进 SOC 电荷计量，不乘端口功率（Q5 红线，避免 double-count）；
% ASSUMED_Bat_Eff_* 与本块无关（仅 ECMS k_eq 内部口径）。

persistent V_1
if isempty(V_1)
    V_1 = 0;    % 极化电压初值 [V]（isempty 初始化）
end

% ---- 1) SOC-LUT（linear 插值 + 域外 clamp，禁止外推；九节点冻结事实源）----
soc_lut = min(max(SOC, Bat_SOC_LUT_nodes(1)), Bat_SOC_LUT_nodes(end));
if SOC > Bat_SOC_LUT_nodes(end)
    ecm_lut_boundary_flag = 1;    % SOC ∈ (0.9, 0.95]：用 0.9 节点值
else
    ecm_lut_boundary_flag = 0;
end
OCV = interp1(Bat_SOC_LUT_nodes, Bat_OCV_LUT_V, soc_lut, 'linear');
R_0 = interp1(Bat_SOC_LUT_nodes, Bat_R0_LUT_ohm, soc_lut, 'linear');
R_1 = interp1(Bat_SOC_LUT_nodes, Bat_R1_LUT_ohm, soc_lut, 'linear');
C_1 = interp1(Bat_SOC_LUT_nodes, Bat_C1_LUT_F, soc_lut, 'linear');

% ---- 2) SOP 四约束（内联自 +model/battery_sop_limits.m，保持一致）----
% 本地映射：OCV_V=OCV（LUT）、V1_V=V_1（persistent 预更新值）、
% [T-013 裁决 2026-09-04] 充放电共用 R_0(SOC)：charging gain ×1.15 无具体文献/实验
% 支撑（顾问表 v1 仅表注一行，Tran 2021 HPPC 未单列充电拟合），暂不人为引入；
% Bat_R0_chg_mult 置 1.0，待真实 BMS 数据后重评。 R0_chg_ohm = R_0 * Bat_R0_chg_mult;
OCV_V = OCV;
V1_V = V_1;
R0_dis_ohm = R_0;
R0_chg_ohm = R_0 * Bat_R0_chg_mult;

% ---- V_oc_est：状态量开路估计（OCV 与 V1 均为状态量，无代数依赖；OQ-9 语义）----
V_oc_est = OCV_V - V1_V;

% ---- 约束 1：P_current（电流 surrogate 上限，bus-side，design §4.6 原式）----
P_current_dis = Bat_I_limit_surrogate_A * V_oc_est / eta_dcdc / 1000;   % kW
P_current_chg = Bat_I_limit_surrogate_A * V_oc_est * eta_dcdc / 1000;   % kW

% ---- 约束 2：P_voltage（端子电压边界反解电流上限，bus-side）----
% 放电：V_t >= V_min 反解 I 上限；端子电压取 max(V_t, V_min) 保证不跌破 V_min
I_vmax = max(V_oc_est - Bat_V_min_V, 0) / max(R0_dis_ohm, 1e-12);
V_t_dis_lim = max(V_oc_est - I_vmax * R0_dis_ohm, Bat_V_min_V);
P_voltage_dis = I_vmax * V_t_dis_lim / eta_dcdc / 1000;                 % kW
% 充电：V_t <= V_max 反解电流上限（I_vmin <= 0）；V_oc_est >= V_max 时 I_vmin=0
% （P_chg=0：开路估计已到上限，不再允许充电）
I_vmin = -max(Bat_V_max_V - V_oc_est, 0) / max(R0_chg_ohm, 1e-12);      % <= 0
V_t_chg_lim = min(V_oc_est - I_vmin * R0_chg_ohm, Bat_V_max_V);
P_voltage_chg = max(abs(I_vmin) * V_t_chg_lim * eta_dcdc / 1000, 0);    % kW，clamp >= 0

% ---- 约束 3：P_SOC（沿用现有降额族；满刻度 = Bat_P_conv_bus_max_kW）----
% 放电：SOC <= DisDerate_Start(0.25) 线性降额 -> SOC_min(0.10) 归零
if SOC <= SOC_min
    P_soc_dis = 0;
    soc_derate_dis = 1;
elseif SOC <= SOC_DisDerate_Start
    P_soc_dis = Bat_P_conv_bus_max_kW * (SOC - SOC_min) / ...
        (SOC_DisDerate_Start - SOC_min);
    soc_derate_dis = 1;
else
    P_soc_dis = Bat_P_conv_bus_max_kW;    % 降额带外：非绑定（与约束 4 同值）
    soc_derate_dis = 0;
end
% 充电：SOC >= ChgDerate_Start(0.90) 线性降额 -> SOC_max(0.95) 归零
if SOC >= SOC_max
    P_soc_chg = 0;
    soc_derate_chg = 1;
elseif SOC >= SOC_ChgDerate_Start
    P_soc_chg = Bat_P_conv_bus_max_kW * (SOC_max - SOC) / ...
        (SOC_max - SOC_ChgDerate_Start);
    soc_derate_chg = 1;
else
    P_soc_chg = Bat_P_conv_bus_max_kW;    % 降额带外：非绑定（与约束 4 同值）
    soc_derate_chg = 0;
end

% ---- 约束 4：P_converter（DC/DC 母线侧图纸额定，bus-side；OQ-9 冻结）----
P_converter = Bat_P_conv_bus_max_kW;

% ---- 四约束取最小（可用功率非负：防退化状态产生负可用功率）----
P_dis_bus_kW = max(min(min(P_current_dis, P_voltage_dis), ...
    min(P_soc_dis, P_converter)), 0);
P_chg_bus_kW = max(min(min(P_current_chg, P_voltage_chg), ...
    min(P_soc_chg, P_converter)), 0);

flags = struct('soc_derate_dis', soc_derate_dis, 'soc_derate_chg', soc_derate_chg);

P_dis_avail_kW = P_dis_bus_kW;
P_chg_avail_kW = P_chg_bus_kW;

% ---- 3) droop 请求 clamp（bus-side；SOP 上/下界，取代旧 lo_clamp/hi_clamp）----
P_bus_kW = min(max(P_droop_kW, -P_chg_avail_kW), P_dis_avail_kW);

% ---- 4) 端子换算（方向感知 DC/DC 效率；×1000 转 W；OQ-9：1050 kW = bus-side）----
if P_bus_kW > 0
    P_t_W = P_bus_kW * 1000 / eta_dcdc;    % 放电：P_t = P_bus/eta
else
    P_t_W = P_bus_kW * 1000 * eta_dcdc;    % 充电：P_t = P_bus*eta
end

% ---- 5) 方向感知 R_0（HPPC surrogate：充电方向内阻 ×Bat_R0_chg_mult）----
if P_t_W >= 0
    R0_eff = R_0;
else
    R0_eff = R_0 * Bat_R0_chg_mult;
end

% ---- 6) 解析求 I（OQ-9 二次式数值稳定形式，无迭代、无代数环）----
battery_power_limited = 0;
battery_discriminant_limit = 0;
E_oc = OCV - V_1;
if E_oc < 1e-3
    % NaN/Inf 防护：E 退化（≈0）→ 走 D<0 power-limit 分支语义
    P_t_act_W = E_oc^2 / (4 * R0_eff);
    I = E_oc / (2 * R0_eff);
    battery_power_limited = 1;
    battery_discriminant_limit = 1;
else
    D = E_oc^2 - 4 * R0_eff * P_t_W;
    if D >= 0
        % 小电流物理根（数值稳定形式，避免 E-sqrt(D) 大数相减）
        P_t_act_W = P_t_W;
        I = 2 * P_t_W / (E_oc + sqrt(D));
    else
        % 判别式 < 0：请求超过 ECM 状态物理极限 P_max_R = E^2/(4*R0)
        % （power-limit semantics：取 P_actual = P_max_R 重算电流；
        %   D_act = E^2 - 4*R0*P_max_R = 0 → I = 2*P_max_R/E = E/(2*R0)）
        P_t_act_W = E_oc^2 / (4 * R0_eff);
        I = E_oc / (2 * R0_eff);
        battery_power_limited = 1;
        battery_discriminant_limit = 1;
    end
end

% ---- 7) 端电压 V_t（= V_bat 输出；用预更新 V_1，状态语义）----
V_t = OCV - I * R0_eff - V_1;

% ---- 8) 极化状态 Euler 步进（persistent；0.01 s 离散，供下一步使用）----
V_1 = V_1 + dt * (-V_1 / (R_1 * C_1) + I / C_1);

% ---- 9) SOC 电荷积分速率（输出给外部 Integrator；eta_coul 仅进 SOC 计量）----
% 放电：dSOC = -I*dt/Q_nom；充电：dSOC = -eta_coul*I*dt/Q_nom（I<0 为正，入账打折）
if I >= 0
    dSOC_dt = -I / (3600 * Bat_Q_nom_Ah);
else
    dSOC_dt = -Bat_eta_coul * I / (3600 * Bat_Q_nom_Ah);
end

% ---- 10) 实际端口功率输出（clamp 后再经 D<0 修正的值）----
if battery_power_limited == 1
    % D<0 仅可能发生在放电方向（充电时 D = E^2 + 4*R0*|P_t| > 0 恒成立）；
    % E 退化防护分支的 P_t_act >= 0 亦按放电口径反算 bus-side
    P_bat_bus_kW = P_t_act_W * eta_dcdc / 1000;
else
    P_bat_bus_kW = P_bus_kW;    % 请求经 SOP clamp 后被 ECM 完全满足
end
SOC_out = SOC;
V_bat_V = V_t;
I_bat_A = I;
end

== matlab function HybridShip_ModelE_PlantStepE_Stream/08_Undervolt_Derate/derate_fn ==
  data: V input; f output; CCS_Vdc_Steady_Band parameter; CCS_Vdc_Transient_Band parameter
function f = derate_fn(V, CCS_Vdc_Steady_Band, CCS_Vdc_Transient_Band)
% 欠压降额系数：CCS 稳态下限以上 f=1，线性降至瞬态下限 f=0
v_lo = CCS_Vdc_Transient_Band(1);
v_hi = CCS_Vdc_Steady_Band(1);
f = min(max((V - v_lo) / (v_hi - v_lo), 0), 1);
end

== matlab function HybridShip_ModelE_PlantStepE_Stream/10_Fuel_Consumption/fuel_model ==
  data: P1_kW input; fuel_rate_1_kg_s output; state1 input; P2_kW input; state2 input; fuel_rate_2_kg_s output; fuel_rate_total_kg_s output; DG_BSFC_P_kW parameter size=5; DG_BSFC_gkWh parameter size=5; DG_C_start_kg parameter; DG_t_starting_s parameter; DG_t_sync_s parameter
function [fuel_rate_1_kg_s, fuel_rate_2_kg_s, fuel_rate_total_kg_s] = FuelModelE(...
    P1_kW, state1, P2_kW, state2, ...
    DG_BSFC_P_kW, DG_BSFC_gkWh, DG_C_start_kg, DG_t_starting_s, DG_t_sync_s)
%#codegen
% FuelModelE：per-genset 燃油模型（Model E, FR-420, design 4.4, OQ-6 方案 A）
%   每机组独立计量，total = rate_1 + rate_2 [kg/s]：
%   ON(state=3)：rate = P * BSFC_pchip(clamp(P,[125,500])) / 3.6e6
%     BSFC LUT 只在 ON 态使用；P<P_min 的爬坡过渡段 clamp 到下节点(125)值查表——
%     不外推、非零；registered surrogate：过渡段怠速油耗未计（与 COOLDOWN 同类局限）；
%     正常下界不可达（由 Plant clamp 保证），此处为防御性 clamp。
%   STARTING/SYNC(state=1|2)：rate = C_start/(t_starting+t_sync)（0.6/30=0.02 kg/s，
%     30 s 积分恰为 C_start——启动燃油只算一次、均摊实现，禁止与 ON 态双算）。
%   OFF/COOLDOWN(state=0|4)：rate = 0（COOLDOWN 怠速油耗未计为 registered 局限）。
fuel_rate_1_kg_s = unit_fuel_rate(P1_kW, state1, DG_BSFC_P_kW, DG_BSFC_gkWh, ...
    DG_C_start_kg, DG_t_starting_s, DG_t_sync_s);
fuel_rate_2_kg_s = unit_fuel_rate(P2_kW, state2, DG_BSFC_P_kW, DG_BSFC_gkWh, ...
    DG_C_start_kg, DG_t_starting_s, DG_t_sync_s);
fuel_rate_total_kg_s = fuel_rate_1_kg_s + fuel_rate_2_kg_s;
end

function r = unit_fuel_rate(P_kW, st, P_bp, g_kWh, C_start_kg, t_starting_s, t_sync_s)
% 单机组瞬时燃油率 [kg/s]（state: 0=OFF 1=STARTING 2=SYNC 3=ON 4=COOLDOWN）
if st == 3
    % ON：防御性 clamp 到 BSFC 定义域节点 [125,500]（禁止 P<P_min 外推）
    P_c = min(max(P_kW, P_bp(1)), P_bp(end));
    bsfc_g_kWh = interp1(P_bp, g_kWh, P_c, 'pchip');
    r = P_kW * bsfc_g_kWh / 3.6e6;   % kW × g/kWh = g/h → /3.6e6 → kg/s
elseif st == 1 || st == 2
    % STARTING/SYNC：启动燃油均摊（只算一次，方案 A event-level surrogate）
    r = C_start_kg / (t_starting_s + t_sync_s);
else
    % OFF / COOLDOWN：怠速油耗未计（registered 局限）
    r = 0;
end
end

== matlab function HybridShip_ModelE_PlantStepE_Stream/13_DC_Bus/dVdt ==
  data: P_res_kW input; dv output; V input; ASSUMED_C_bus parameter; ASSUMED_V_floor parameter
function dv = dVdt(P_res_kW, V, ASSUMED_C_bus, ASSUMED_V_floor)
% 母线电压动态：C*V*dV/dt = P_res（kW -> W 换算，V_floor 除法保护）
dv = P_res_kW * 1000 / (ASSUMED_C_bus * max(V, ASSUMED_V_floor));
end

== matlab function HybridShip_ModelE_PlantStepE_Stream/15_Bus_Voltage_Monitor/ccs_check ==
  data: V input; al_s output; al_t output; CCS_Vdc_Steady_Band parameter; CCS_Vdc_Transient_Band parameter
function [al_s, al_t] = ccs_check(V, CCS_Vdc_Steady_Band, CCS_Vdc_Transient_Band)
% CCS 2026 电能质量判定：稳态带 -10%/+6%，瞬态带 -20%/+7%
al_s = double(V < CCS_Vdc_Steady_Band(1) || V > CCS_Vdc_Steady_Band(2));
al_t = double(V < CCS_Vdc_Transient_Band(1) || V > CCS_Vdc_Transient_Band(2));
end

== matlab function HybridShip_ModelE_PlantStepE_Stream/01_Operator_Interface/current_profile ==
  data: x input; vc output; t input; mode input; kx input; kv input; v_def input; tt input; tv input
function vc = current_profile(x, t, mode, kx, kv, v_def, tt, tv)
% 水流速度剖面：mode=0 按里程节点分段线性（既有；负=逆水，正=顺水，节点 -1 结束）
% mode=1 按时间节点分段恒定（S20：仅段 9 逆水 -1 m/s，其余 0）
if mode > 0.5
    vc = v_def;
    if tt(1) < 0
        return;
    end
    if t <= tt(1)
        vc = tv(1);
        return;
    end
    for k = 1:numel(tt)-1
        if t < tt(k+1)
            vc = tv(k);
            return;
        end
    end
    vc = tv(end);
    return;
end
vc = v_def;
if kx(1) < 0
    return;
end
if x <= kx(1)
    vc = kv(1);
    return;
end
for k = 1:3
    if kx(k+1) < 0
        vc = kv(k);
        return;
    end
    if x <= kx(k+1)
        w = (x - kx(k)) / max(kx(k+1) - kx(k), 1e-6);
        vc = kv(k) + w * (kv(k+1) - kv(k));
        return;
    end
end
vc = kv(4);
end

== matlab function HybridShip_ModelE_PlantStepE_Stream/01_Operator_Interface/v_cmd_profile ==
  data: x input; v output; t input; mode input; kx input; kv input; v_def input; tt input; tv input
function v = v_cmd_profile(x, t, mode, kx, kv, v_def, tt, tv)
% 目标航速剖面：mode=0 距离节点分段线性（既有语义）；mode=1 时间节点分段恒定（S20，design §2.1）
% 时间模式过渡由下游 Rate Limiter 按 SCN.accel/decel_ramp_mps2 平滑（以限幅器为准）
if mode > 0.5
    v = v_def;
    if tt(1) < 0
        return;
    end
    if t <= tt(1)
        v = tv(1);
        return;
    end
    for k = 1:numel(tt)-1
        if t < tt(k+1)
            v = tv(k);
            return;
        end
    end
    v = tv(end);
    return;
end
v = v_def;
if kx(1) < 0
    return;
end
if x <= kx(1)
    v = kv(1);
    return;
end
for k = 1:5
    if kx(k+1) < 0
        v = kv(k);
        return;
    end
    if x <= kx(k+1)
        w = (x - kx(k)) / max(kx(k+1) - kx(k), 1e-6);
        v = kv(k) + w * (kv(k+1) - kv(k));
        return;
    end
end
v = kv(6);
end

== matlab function HybridShip_ModelE_PlantStepE_Stream/01_Operator_Interface/resist_profile ==
  data: x input; m output; profile input; pos input; amp input; rampT input; bands input; v_target input
function m = resist_profile(x, profile, pos, amp, rampT, bands, v_target)
% 阻力倍率剖面（距离触发，x 平滑过渡；无状态，适合连续采样）
% 过渡带宽度 = v_target * rampT（约 10~20 s 对应距离）；bands: 4x3 [起点 终点 幅值]，起点<0 结束
dx = v_target * max(rampT, 1e-6);
r = min(max((x - pos) / max(dx, 1e-6), 0), 1);
switch profile
    case 0
        m = 1;
    case 1
        m = 1 + amp * r;
    case 2
        m = 1 + amp * r;
    case 3
        if x >= pos, m = 1 + amp; else, m = 1; end
    case 4
        m = 1;
        for k = 1:4
            xs = bands(k, 1);
            if xs < 0
                break;
            end
            xe = bands(k, 2);
            a = bands(k, 3);
            r_up = min(max((x - xs) / max(dx, 1e-6), 0), 1);
            r_dn = min(max((x - xe) / max(dx, 1e-6), 0), 1);
            m = m + a * (r_up - r_dn);
        end
    otherwise
        m = 1;
end
m = max(m, 0.05);
end

== matlab function HybridShip_ModelE_PlantStepE_Stream/03_Propulsion_Plant/Propeller_Hydrodynamics ==
  data: n_prop_rpm input; F_prop_eff output; V_ship_mps input; V_current_mps input; w_signal input; Q_prop output; P_hydro_kW output; V_A output; K_Fw parameter; K_Fv parameter; K_Qw parameter; K_Qv parameter
function [F_prop_eff, Q_prop, P_hydro_kW, V_A] = PropellerHydroSimpleE(...
    n_prop_rpm, V_ship_mps, V_current_mps, w_signal, K_Fw, K_Fv, K_Qw, K_Qv)
% 简化螺旋桨水动力模型（Model E，T-005：与 legacy PropellerHydroSimple 完全同构）
% 唯一差异：wake_fraction 由 Parameter 改为输入信号 w_signal（w(H/T) 来自 Wake_vs_HT）
% 螺旋桨 D、K_T/K_Q、P/D 保持 INTENTIONALLY UNRESOLVED（FR-417），不得填入借用值
omega = n_prop_rpm * pi / 30;
V_rel = V_ship_mps - V_current_mps;
V_A = (1 - w_signal) * V_rel;
F_prop_eff = K_Fw * omega * abs(omega) - K_Fv * V_A * abs(V_A);
Q_prop = K_Qw * omega * abs(omega) - K_Qv * V_A * abs(V_A);
P_hydro_kW = Q_prop * omega / 1000;
end
